simulink model "EINT_RL_closed_loop_2"  (R2026b)
settings: Solver=FixedStepAuto  StopTime=T_end  FixedStep=Ts
values from neighbouring files (symbols this model uses):
  Ts = 0.05    [EINT_RL_eval.m]    (also in EINT_RL_eval2.m)
settings Model: Creator=etienne  LastModifiedBy=hp
settings RTWCC: GPUComputeCapability=5.0

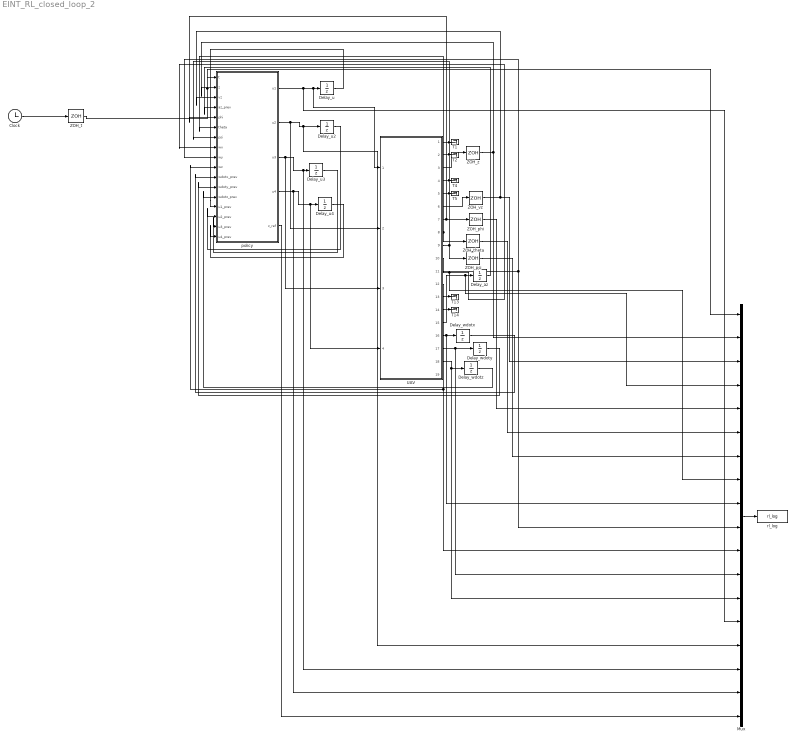
== system EINT_RL_closed_loop_2 ==
  Clock : Clock
  Delay_az : UnitDelay  SampleTime=Ts
  Delay_u{,2..4} (4 alike) : UnitDelay  SampleTime=Ts
  Delay_wdotx : UnitDelay  SampleTime=Ts
  Delay_wdoty : UnitDelay  SampleTime=Ts
  Delay_wdotz : UnitDelay  SampleTime=Ts
  Mux : Mux  Inputs=18
  T{1..2,4..5,13..14} (6 alike) : Terminator
  UAV : Subsystem  ReferencedSubsystem=UAV_model
  ZOH_phi : ZeroOrderHold  SampleTime=Ts
  ZOH_psi : ZeroOrderHold  SampleTime=Ts
  ZOH_t : ZeroOrderHold  SampleTime=Ts
  ZOH_theta : ZeroOrderHold  SampleTime=Ts
  ZOH_vz : ZeroOrderHold  SampleTime=Ts
  ZOH_z : ZeroOrderHold  SampleTime=Ts
  policy : MATLAB Function  TreatAsAtomicUnit=on
  rl_log : ToWorkspace  VariableName=rl_log  SampleTime=Ts
  wires:
  Clock/1 -> ZOH_t/1
  UAV/3 -> ZOH_z/1
  UAV/6 -> ZOH_vz/1
  UAV/15 -> Mux/4, Delay_az/1
  ZOH_t/1 -> Mux/1, policy/1(t)
  ZOH_z/1 -> Mux/2, policy/2(z)
  ZOH_vz/1 -> Mux/3, policy/3(vz)
  Delay_az/1 -> policy/4(az_prev)
  policy/1(u1) -> Mux/14, UAV/1, Delay_u/1
  UAV/1 -> T1/1
  UAV/2 -> T2/1
  UAV/4 -> T4/1
  UAV/5 -> T5/1
  UAV/13 -> T13/1
  UAV/14 -> T14/1
  UAV/16 -> Delay_wdotx/1, Mux/9
  policy/5(z_ref) -> Mux/18
  Mux/1 -> rl_log/1
  UAV/17 -> Mux/12, Delay_wdoty/1
  UAV/18 -> Mux/13, Delay_wdotz/1
  UAV/7 -> ZOH_phi/1, policy/5(phi)
  ZOH_phi/1 -> Mux/5
  UAV/8 -> policy/6(theta), ZOH_theta/1
  ZOH_theta/1 -> Mux/6
  UAV/9 -> policy/7(psi), ZOH_psi/1
  ZOH_psi/1 -> Mux/7
  Delay_wdotz/1 -> policy/13(wdotz_prev)
  Delay_wdoty/1 -> policy/12(wdoty_prev)
  Delay_wdotx/1 -> policy/11(wdotx_prev)
  UAV/10 -> policy/8(wx), Mux/8
  UAV/11 -> policy/9(wy), Mux/10
  UAV/12 -> policy/10(wz), Mux/11
  policy/4(u4) -> Mux/17, UAV/4, Delay_u4/1
  policy/3(u3) -> UAV/3, Mux/16, Delay_u3/1
  policy/2(u2) -> UAV/2, Mux/15, Delay_u2/1
  Delay_u4/1 -> policy/17(u4_prev)
  Delay_u3/1 -> policy/16(u3_prev)
  Delay_u2/1 -> policy/15(u2_prev)
  Delay_u/1 -> policy/14(u1_prev)

== matlab function EINT_RL_closed_loop_2/policy ==
  data: t input; u1 output; u2 output; u3 output; u4 output; z input; vz input; az_prev input; phi input; theta input; psi input; wx input; wy input; wz input; wdotx_prev input; wdoty_prev input; wdotz_prev input; u1_prev input; z_ref output; u2_prev input; u3_prev input; u4_prev input
function [u1, u2, u3, u4, z_ref] = policy(t, z, vz, az_prev,phi, theta, psi,wx,wy,wz,wdotx_prev,wdoty_prev,wdotz_prev, u1_prev, u2_prev,u3_prev, u4_prev)
coder.extrinsic('rl_controller2');
u1= 0;
u2= 0;
u3= 0;
u4= 0;
z_ref = 0;
[u1, u2, u3, u4, z_ref] = rl_controller2(t, z, vz, az_prev,phi, theta, psi,wx,wy,wz,wdotx_prev,wdoty_prev,wdotz_prev, u1_prev, u2_prev,u3_prev, u4_prev);
